simulink model "PMSG_WECS_blocks"  (R2024b)
settings: Solver=ode4  StartTime=0.0  StopTime=Tend  FixedStep=Ts  RelTol=1e-3
InitFcn:
  | %% Parameters of the Simulink model PMSG_WECS_blocks (run automatically by InitFcn)
  | % Scenario selection (can be set in the Command Window before sim):
  | %   scenario = 'step' | 'nominal' | 'robust' ;  useANN = 1 | 0
  | if ~exist('scenario', 'var'), scenario = 'robust'; end
  | if ~exist('useANN', 'var'),   useANN = 1;         end
  | %% Turbine
  | rho = 1.225;  R = 40;  Pn = 2e6;  Wn = 2.23;  Tn = Pn/Wn;
  | J = 2.8e6;  B = 1e3;  lopt = 8.1;  vn = Wn*R/lopt;
  | lam_tab = linspace(1, 16, 301);
  | li_tab  = 1./(1./lam_tab - 0.035);
  | cp_tab  = max(0.5176*(116./li_tab - 5).*exp(-21./li_tab) + 0.0068*lam_tab, 0);
  | %% PMSG (Hasan & Shatil, AJSE 2021, Table I)
  | p = 26;  Rs = 0.78e-3;  Ls = 1.57e-3;  psi = 9.18;
  | %% DC link, filter, grid
  | C = 20e-3;  Vdcr = 1200;  Vgm = 690*sqrt(2/3);  wg = 2*pi*50;
  | Lf = 0.15e-3;  Rf = 2e-3;  fsw = 2160;
  | In = Pn/(1.5*Vgm);  Temax = 1.2*Tn;  Igmax = 1.3*In;  Wmin = 0.5*Wn;  Wmax = Wn;
  | %% Sampling and simulation
  | Ts = 1/(2*fsw);  Tend = 40;  Tlog = 10*Ts;
  | %% Wind
  | Vm = 8.5;  Aw = [1.5 0.2 0.3];  fw = [0.03 0.16 0.17];
  | sig_t = 0.5;  tau_t = 1.5;  seed = 12345;  tau_a = 1.0;
  | Tn_w = 4*Ts;  an = exp(-Tn_w/tau_t);  gn = sqrt(1 - an^2)*sig_t;
  | %% Control
  | wr = 1;  wW = 2;  k11 = 2*wW;  k12 = wW^2;  wv = 60;  k21 = 2*wv;  k22 = wv^2;
  | wi = 500;  Ra = 2*wi*Ls - Rs;  Ki = wi^2*Ls;  Rb = 2*wi*Lf - Rf;  Kig = wi^2*Lf;
  | taud = 2e-3;  kI = k12*(1 - useANN);
  | [c1g, c2g] = meshgrid(linspace(0.5, 1.1, 5), linspace(0.5, 1.1, 5));
  | c1 = c1g(:);  c2 = c2g(:);  b = 0.15;  Gam = 1e7;  sig = 0.02;
  | %% True plant (robustness scenario: parameter mismatch + 50 % grid voltage dip)
  | kTw = 1;  Jt = J;  Rst = Rs;  Lst = Ls;  psit = psi;  Rft = Rf;  Lft = Lf;  Bt = B;
  | windStep = 0;  v0 = Vm;  kdip = 0;  tdip = 25;  ddip = 0.15;
  | switch scenario
  |   case 'step'
  |     windStep = 1;  v0 = 9;
  |   case 'robust'
  |     kTw = 1.10;  Jt = 1.2*J;  Rst = 1.5*Rs;  Lst = 1.2*Ls;  psit = 0.95*psi;
  |     Rft = 1.5*Rf;  Lft = 1.25*Lf;  kdip = 0.5;
  | end
  | %% Initial equilibrium (MPPT at v0, isd = 0, unity power factor)
  | cpf  = @(l) max(0.5176*(116./(1./(1./l - 0.035)) - 5).*exp(-21./(1./(1./l - 0.035))) + 0.0068*l, 0);
  | aero = @(W, v) 0.5*rho*pi*R^2*cpf(W*R/v)*v^3/W;
  | W0   = min(max(lopt*v0/R, Wmin), Wmax);
  | isq0 = -(kTw*aero(W0, v0) - Bt*W0)/(1.5*p*psit);
  | we0  = p*W0;
  | us0  = [-we0*Lst*isq0; Rst*isq0 + we0*psit];
  | Pdc0 = -1.5*us0(2)*isq0;
  | igd0 = (-Vgm + sqrt(Vgm^2 + 4*Rft*Pdc0/1.5))/(2*Rft);
  | ui0  = [Rft*igd0 + Vgm; wg*Lft*igd0];
  | Te0c = 1.5*p*psi*isq0;
  | zW0  = (B*W0 - aero(W0, v0) - Te0c)/(J*k12) * (1 - useANN);
values from neighbouring files (symbols this model uses):
  useANN = 1 | 0'    [PMSG_WECS_simulink.m]
undefined symbols (not defined in the file or in its folder): DiscIntNeverNeededParam
settings Model: Creator=WINDOWS  LastModifiedBy=WINDOWS

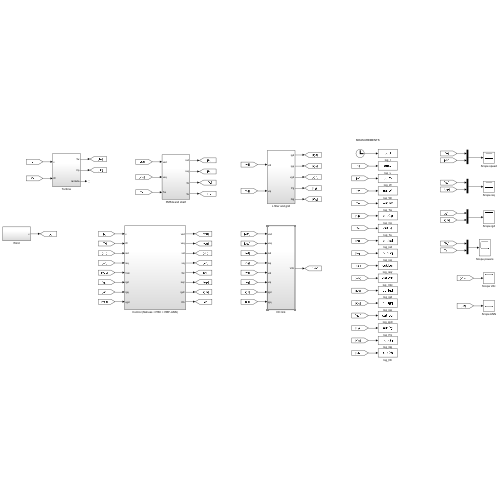
[thumbnail: Simulink's stored preview of the top-level diagram]
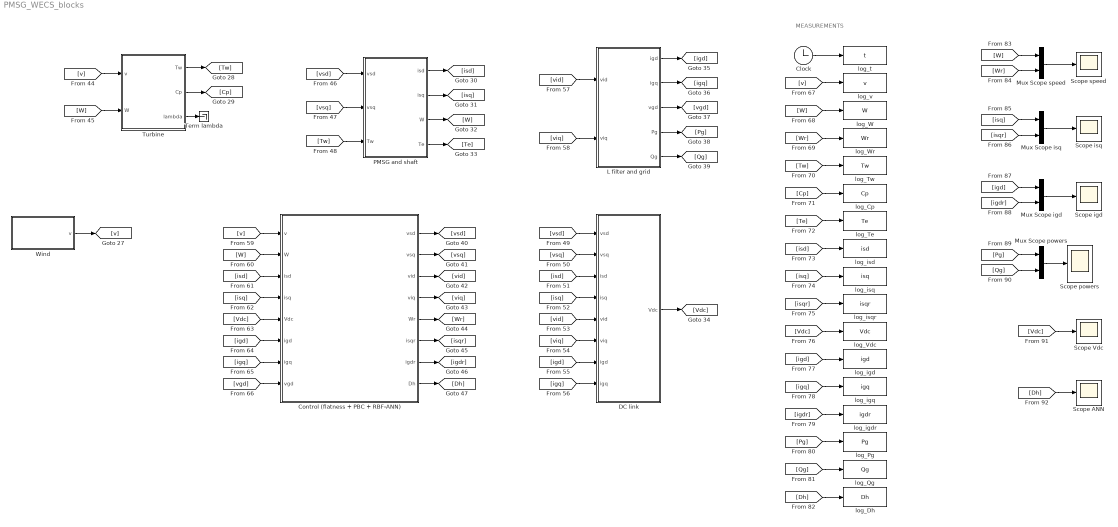
== system PMSG_WECS_blocks ==
  note: MEASUREMENTS
  Clock : Clock
  Control (flatness + PBC + RBF-ANN) : Subsystem
  DC link : Subsystem
  L filter and grid : Subsystem
  Mux Scope igd : Mux  Inputs=2
  Mux Scope isq : Mux  Inputs=2
  Mux Scope powers : Mux  Inputs=2
  Mux Scope speed : Mux  Inputs=2
  PMSG and shaft : Subsystem
  Scope ANN : Scope
  Scope Vdc : Scope
  Scope igd : Scope
  Scope isq : Scope
  Scope powers : Scope
  Scope speed : Scope
  Term lambda : Terminator
  Turbine : Subsystem
  Wind : Subsystem
  log_Cp : ToWorkspace  VariableName=Cp  SampleTime=Tlog
  log_Dh : ToWorkspace  VariableName=Dh  SampleTime=Tlog
  log_Pg : ToWorkspace  VariableName=Pg  SampleTime=Tlog
  log_Qg : ToWorkspace  VariableName=Qg  SampleTime=Tlog
  log_Te : ToWorkspace  VariableName=Te  SampleTime=Tlog
  log_Tw : ToWorkspace  VariableName=Tw  SampleTime=Tlog
  log_Vdc : ToWorkspace  VariableName=Vdc  SampleTime=Tlog
  log_W : ToWorkspace  VariableName=W  SampleTime=Tlog
  log_Wr : ToWorkspace  VariableName=Wr  SampleTime=Tlog
  log_igd : ToWorkspace  VariableName=igd  SampleTime=Tlog
  log_igdr : ToWorkspace  VariableName=igdr  SampleTime=Tlog
  log_igq : ToWorkspace  VariableName=igq  SampleTime=Tlog
  log_isd : ToWorkspace  VariableName=isd  SampleTime=Tlog
  log_isq : ToWorkspace  VariableName=isq  SampleTime=Tlog
  log_isqr : ToWorkspace  VariableName=isqr  SampleTime=Tlog
  log_t : ToWorkspace  VariableName=t  SampleTime=Tlog
  log_v : ToWorkspace  VariableName=v  SampleTime=Tlog
  wires:
  Wind/1(v) -> [v]
  Turbine/1(Tw) -> [Tw]
  Turbine/2(Cp) -> [Cp]
  PMSG and shaft/1(isd) -> [isd]
  PMSG and shaft/2(isq) -> [isq]
  PMSG and shaft/3(W) -> [W]
  PMSG and shaft/4(Te) -> [Te]
  DC link/1(Vdc) -> [Vdc]
  L filter and grid/1(igd) -> [igd]
  L filter and grid/2(igq) -> [igq]
  L filter and grid/3(vgd) -> [vgd]
  L filter and grid/4(Pg) -> [Pg]
  L filter and grid/5(Qg) -> [Qg]
  Control (flatness + PBC + RBF-ANN)/1(vsd) -> [vsd]
  Control (flatness + PBC + RBF-ANN)/2(vsq) -> [vsq]
  Control (flatness + PBC + RBF-ANN)/3(vid) -> [vid]
  Control (flatness + PBC + RBF-ANN)/4(viq) -> [viq]
  Control (flatness + PBC + RBF-ANN)/5(Wr) -> [Wr]
  Control (flatness + PBC + RBF-ANN)/6(isqr) -> [isqr]
  Control (flatness + PBC + RBF-ANN)/7(igdr) -> [igdr]
  Control (flatness + PBC + RBF-ANN)/8(Dh) -> [Dh]
  Turbine/3(lambda) -> Term lambda/1
  [v] -> Turbine/1(v)
  [W] -> Turbine/2(W)
  [vsd] -> PMSG and shaft/1(vsd)
  [vsq] -> PMSG and shaft/2(vsq)
  [Tw] -> PMSG and shaft/3(Tw)
  [vsd] -> DC link/1(vsd)
  [vsq] -> DC link/2(vsq)
  [isd] -> DC link/3(isd)
  [isq] -> DC link/4(isq)
  [vid] -> DC link/5(vid)
  [viq] -> DC link/6(viq)
  [igd] -> DC link/7(igd)
  [igq] -> DC link/8(igq)
  [vid] -> L filter and grid/1(vid)
  [viq] -> L filter and grid/2(viq)
  [v] -> Control (flatness + PBC + RBF-ANN)/1(v)
  [W] -> Control (flatness + PBC + RBF-ANN)/2(W)
  [isd] -> Control (flatness + PBC + RBF-ANN)/3(isd)
  [isq] -> Control (flatness + PBC + RBF-ANN)/4(isq)
  [Vdc] -> Control (flatness + PBC + RBF-ANN)/5(Vdc)
  [igd] -> Control (flatness + PBC + RBF-ANN)/6(igd)
  [igq] -> Control (flatness + PBC + RBF-ANN)/7(igq)
  [vgd] -> Control (flatness + PBC + RBF-ANN)/8(vgd)
  Clock/1 -> log_t/1
  [v] -> log_v/1
  [W] -> log_W/1
  [Wr] -> log_Wr/1
  [Tw] -> log_Tw/1
  [Cp] -> log_Cp/1
  [Te] -> log_Te/1
  [isd] -> log_isd/1
  [isq] -> log_isq/1
  [isqr] -> log_isqr/1
  [Vdc] -> log_Vdc/1
  [igd] -> log_igd/1
  [igq] -> log_igq/1
  [igdr] -> log_igdr/1
  [Pg] -> log_Pg/1
  [Qg] -> log_Qg/1
  [Dh] -> log_Dh/1
  [W] -> Mux Scope speed/1
  [Wr] -> Mux Scope speed/2
  Mux Scope speed/1 -> Scope speed/1
  [isq] -> Mux Scope isq/1
  [isqr] -> Mux Scope isq/2
  Mux Scope isq/1 -> Scope isq/1
  [igd] -> Mux Scope igd/1
  [igdr] -> Mux Scope igd/2
  Mux Scope igd/1 -> Scope igd/1
  [Pg] -> Mux Scope powers/1
  [Qg] -> Mux Scope powers/2
  Mux Scope powers/1 -> Scope powers/1
  [Vdc] -> Scope Vdc/1
  [Dh] -> Scope ANN/1

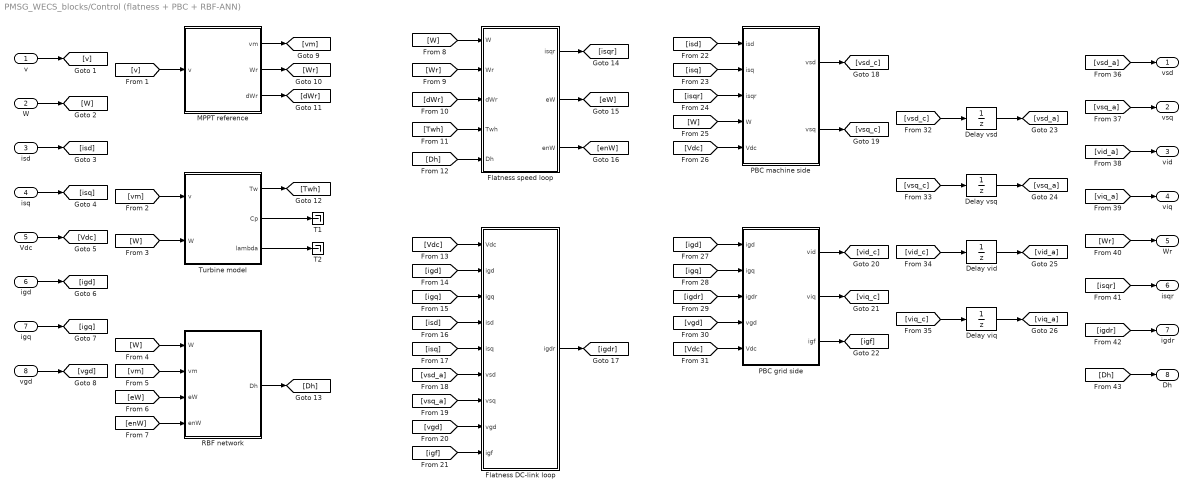
== system PMSG_WECS_blocks/Control (flatness + PBC + RBF-ANN) ==
  v : Inport
  W : Inport  Port=2
  isd : Inport  Port=3
  isq : Inport  Port=4
  Vdc : Inport  Port=5
  igd : Inport  Port=6
  igq : Inport  Port=7
  vgd : Inport  Port=8
  Delay vid : UnitDelay  InitialCondition=ui0(1)  SampleTime=Ts  HasFrameUpgradeWarning=on
  Delay viq : UnitDelay  InitialCondition=ui0(2)  SampleTime=Ts  HasFrameUpgradeWarning=on
  Delay vsd : UnitDelay  InitialCondition=us0(1)  SampleTime=Ts  HasFrameUpgradeWarning=on
  Delay vsq : UnitDelay  InitialCondition=us0(2)  SampleTime=Ts  HasFrameUpgradeWarning=on
  Flatness DC-link loop : Subsystem
  Flatness speed loop : Subsystem
  MPPT reference : Subsystem
  PBC grid side : Subsystem
  PBC machine side : Subsystem
  RBF network : Subsystem
  T1 : Terminator
  T2 : Terminator
  Turbine model : Subsystem
  vsd : Outport
  vsq : Outport  Port=2
  vid : Outport  Port=3
  viq : Outport  Port=4
  Wr : Outport  Port=5
  isqr : Outport  Port=6
  igdr : Outport  Port=7
  Dh : Outport  Port=8
  wires:
  Turbine model/2(Cp) -> T1/1
  Turbine model/3(lambda) -> T2/1
  v/1 -> [v]
  W/1 -> [W]
  isd/1 -> [isd]
  isq/1 -> [isq]
  Vdc/1 -> [Vdc]
  igd/1 -> [igd]
  igq/1 -> [igq]
  vgd/1 -> [vgd]
  MPPT reference/1(vm) -> [vm]
  MPPT reference/2(Wr) -> [Wr]
  MPPT reference/3(dWr) -> [dWr]
  Turbine model/1(Tw) -> [Twh]
  RBF network/1(Dh) -> [Dh]
  Flatness speed loop/1(isqr) -> [isqr]
  Flatness speed loop/2(eW) -> [eW]
  Flatness speed loop/3(enW) -> [enW]
  Flatness DC-link loop/1(igdr) -> [igdr]
  PBC machine side/1(vsd) -> [vsd_c]
  PBC machine side/2(vsq) -> [vsq_c]
  PBC grid side/1(vid) -> [vid_c]
  PBC grid side/2(viq) -> [viq_c]
  PBC grid side/3(igf) -> [igf]
  Delay vsd/1 -> [vsd_a]
  Delay vsq/1 -> [vsq_a]
  Delay vid/1 -> [vid_a]
  Delay viq/1 -> [viq_a]
  [v] -> MPPT reference/1(v)
  [vm] -> Turbine model/1(v)
  [W] -> Turbine model/2(W)
  [W] -> RBF network/1(W)
  [vm] -> RBF network/2(vm)
  [eW] -> RBF network/3(eW)
  [enW] -> RBF network/4(enW)
  [W] -> Flatness speed loop/1(W)
  [Wr] -> Flatness speed loop/2(Wr)
  [dWr] -> Flatness speed loop/3(dWr)
  [Twh] -> Flatness speed loop/4(Twh)
  [Dh] -> Flatness speed loop/5(Dh)
  [Vdc] -> Flatness DC-link loop/1(Vdc)
  [igd] -> Flatness DC-link loop/2(igd)
  [igq] -> Flatness DC-link loop/3(igq)
  [isd] -> Flatness DC-link loop/4(isd)
  [isq] -> Flatness DC-link loop/5(isq)
  [vsd_a] -> Flatness DC-link loop/6(vsd)
  [vsq_a] -> Flatness DC-link loop/7(vsq)
  [vgd] -> Flatness DC-link loop/8(vgd)
  [igf] -> Flatness DC-link loop/9(igf)
  [isd] -> PBC machine side/1(isd)
  [isq] -> PBC machine side/2(isq)
  [isqr] -> PBC machine side/3(isqr)
  [W] -> PBC machine side/4(W)
  [Vdc] -> PBC machine side/5(Vdc)
  [igd] -> PBC grid side/1(igd)
  [igq] -> PBC grid side/2(igq)
  [igdr] -> PBC grid side/3(igdr)
  [vgd] -> PBC grid side/4(vgd)
  [Vdc] -> PBC grid side/5(Vdc)
  [vsd_c] -> Delay vsd/1
  [vsq_c] -> Delay vsq/1
  [vid_c] -> Delay vid/1
  [viq_c] -> Delay viq/1
  [vsd_a] -> vsd/1
  [vsq_a] -> vsq/1
  [vid_a] -> vid/1
  [viq_a] -> viq/1
  [Wr] -> Wr/1
  [isqr] -> isqr/1
  [igdr] -> igdr/1
  [Dh] -> Dh/1

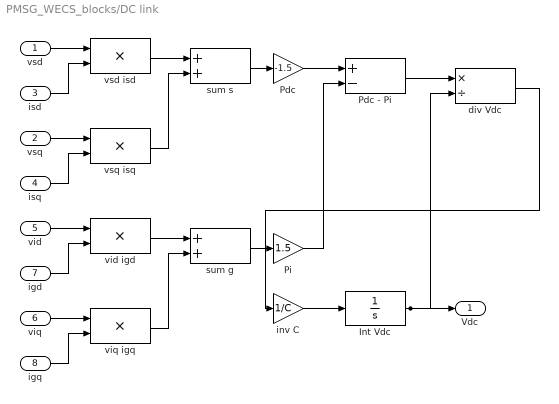
== system PMSG_WECS_blocks/DC link ==
  vsd : Inport
  vsq : Inport  Port=2
  isd : Inport  Port=3
  isq : Inport  Port=4
  vid : Inport  Port=5
  viq : Inport  Port=6
  igd : Inport  Port=7
  igq : Inport  Port=8
  Int Vdc : Integrator  InitialCondition=Vdcr
  Pdc : Gain  Gain=-1.5
  Pdc - Pi : Sum  Inputs=+-
  Pi : Gain  Gain=1.5
  div Vdc : Product  Inputs=*/
  inv C : Gain  Gain=1/C
  sum g : Sum
  sum s : Sum
  vid igd : Product  Inputs=**
  viq igq : Product  Inputs=**
  vsd isd : Product  Inputs=**
  vsq isq : Product  Inputs=**
  Vdc : Outport
  wires:
  vsd/1 -> vsd isd/1
  isd/1 -> vsd isd/2
  vsq/1 -> vsq isq/1
  isq/1 -> vsq isq/2
  viq/1 -> viq igq/1
  vid/1 -> vid igd/1
  igd/1 -> vid igd/2
  igq/1 -> viq igq/2
  vsq isq/1 -> sum s/2
  vsd isd/1 -> sum s/1
  viq igq/1 -> sum g/2
  vid igd/1 -> sum g/1
  sum s/1 -> Pdc/1
  sum g/1 -> Pi/1
  Pdc/1 -> Pdc - Pi/1
  Pi/1 -> Pdc - Pi/2
  inv C/1 -> Int Vdc/1
  Pdc - Pi/1 -> div Vdc/1
  div Vdc/1 -> inv C/1
  Int Vdc/1 -> div Vdc/2, Vdc/1

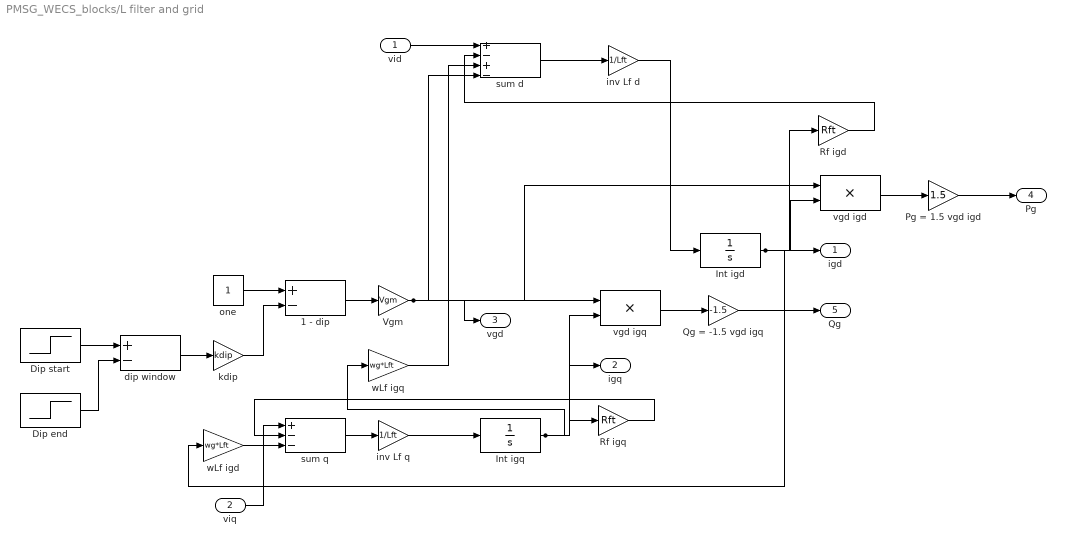
== system PMSG_WECS_blocks/L filter and grid ==
  vid : Inport
  viq : Inport  Port=2
  1 - dip : Sum  Inputs=+-
  Dip end : Step  Time=tdip+ddip  SampleTime=0
  Dip start : Step  Time=tdip  SampleTime=0
  Int igd : Integrator  InitialCondition=igd0
  Int igq : Integrator
  Pg = 1.5 vgd igd : Gain  Gain=1.5
  Qg = -1.5 vgd igq : Gain  Gain=-1.5
  Rf igd : Gain  Gain=Rft
  Rf igq : Gain  Gain=Rft
  Vgm : Gain  Gain=Vgm
  dip window : Sum  Inputs=+-
  inv Lf d : Gain  Gain=1/Lft
  inv Lf q : Gain  Gain=1/Lft
  kdip : Gain  Gain=kdip
  one : Constant
  sum d : Sum  Inputs=+-+-
  sum q : Sum  Inputs=+--
  vgd igd : Product  Inputs=**
  vgd igq : Product  Inputs=**
  wLf igd : Gain  Gain=wg*Lft
  wLf igq : Gain  Gain=wg*Lft
  igd : Outport
  igq : Outport  Port=2
  vgd : Outport  Port=3
  Pg : Outport  Port=4
  Qg : Outport  Port=5
  wires:
  sum q/1 -> inv Lf q/1
  wLf igd/1 -> sum q/3
  Dip start/1 -> dip window/1
  Dip end/1 -> dip window/2
  viq/1 -> sum q/1
  kdip/1 -> 1 - dip/2
  dip window/1 -> kdip/1
  one/1 -> 1 - dip/1
  1 - dip/1 -> Vgm/1
  vid/1 -> sum d/1
  Vgm/1 -> vgd igq/1, vgd/1, sum d/4, vgd igd/1
  sum d/1 -> inv Lf d/1
  wLf igq/1 -> sum d/3
  inv Lf q/1 -> Int igq/1
  Int igq/1 -> wLf igq/1, Rf igq/1, vgd igq/2, igq/1
  inv Lf d/1 -> Int igd/1
  vgd igq/1 -> Qg = -1.5 vgd igq/1
  Rf igq/1 -> sum q/2
  Int igd/1 -> wLf igd/1, Rf igd/1, vgd igd/2, igd/1
  Qg = -1.5 vgd igq/1 -> Qg/1
  Rf igd/1 -> sum d/2
  vgd igd/1 -> Pg = 1.5 vgd igd/1
  Pg = 1.5 vgd igd/1 -> Pg/1

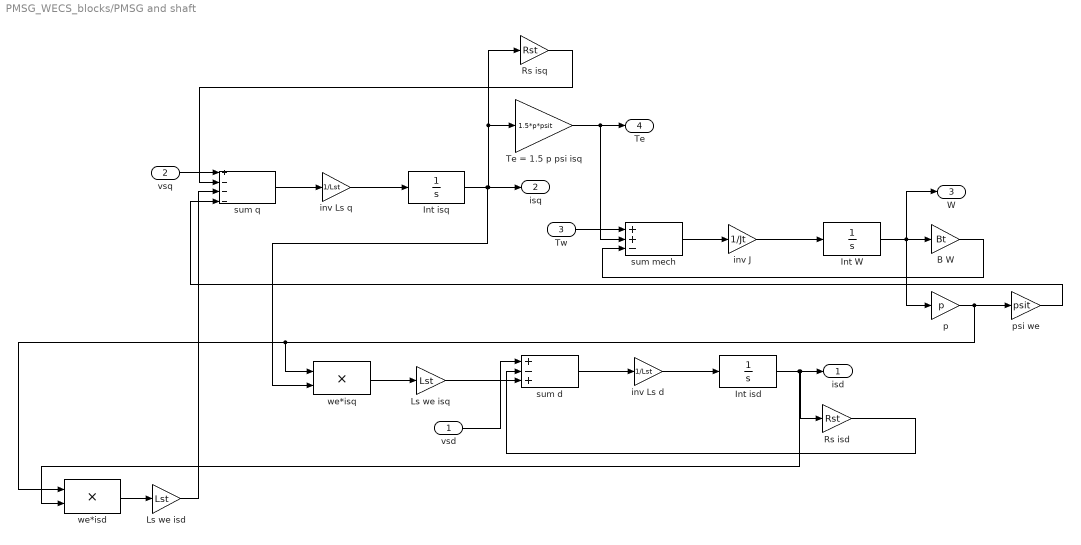
== system PMSG_WECS_blocks/PMSG and shaft ==
  vsd : Inport
  vsq : Inport  Port=2
  Tw : Inport  Port=3
  B W : Gain  Gain=Bt
  Int W : Integrator  InitialCondition=W0
  Int isd : Integrator
  Int isq : Integrator  InitialCondition=isq0
  Ls we isd : Gain  Gain=Lst
  Ls we isq : Gain  Gain=Lst
  Rs isd : Gain  Gain=Rst
  Rs isq : Gain  Gain=Rst
  Te = 1.5 p psi isq : Gain  Gain=1.5*p*psit
  inv J : Gain  Gain=1/Jt
  inv Ls d : Gain  Gain=1/Lst
  inv Ls q : Gain  Gain=1/Lst
  p : Gain  Gain=p
  psi we : Gain  Gain=psit
  sum d : Sum  Inputs=+-+
  sum mech : Sum  Inputs=++-
  sum q : Sum  Inputs=+---
  we*isd : Product  Inputs=**
  we*isq : Product  Inputs=**
  isd : Outport
  isq : Outport  Port=2
  W : Outport  Port=3
  Te : Outport  Port=4
  wires:
  Int isq/1 -> Te = 1.5 p psi isq/1, Rs isq/1, isq/1, we*isq/2
  Int W/1 -> p/1, B W/1, W/1
  Int isd/1 -> Rs isd/1, isd/1, we*isd/2
  we*isd/1 -> Ls we isd/1
  vsq/1 -> sum q/1
  sum q/1 -> inv Ls q/1
  Ls we isd/1 -> sum q/3
  inv Ls q/1 -> Int isq/1
  Ls we isq/1 -> sum d/3
  we*isq/1 -> Ls we isq/1
  vsd/1 -> sum d/1
  Rs isq/1 -> sum q/2
  Te = 1.5 p psi isq/1 -> sum mech/2, Te/1
  Tw/1 -> sum mech/1
  sum d/1 -> inv Ls d/1
  inv J/1 -> Int W/1
  sum mech/1 -> inv J/1
  inv Ls d/1 -> Int isd/1
  Rs isd/1 -> sum d/2
  B W/1 -> sum mech/3
  p/1 -> we*isq/1, we*isd/1, psi we/1
  psi we/1 -> sum q/4

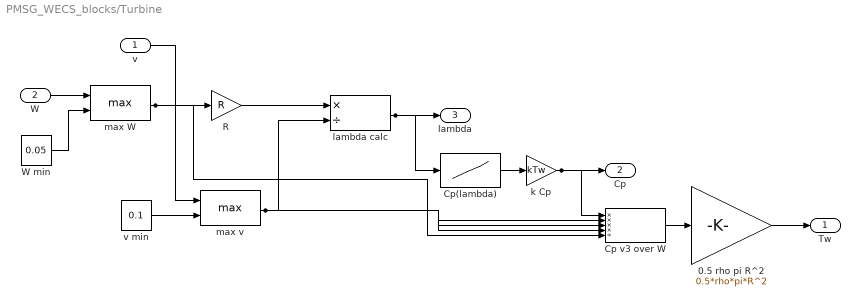
== system PMSG_WECS_blocks/Turbine ==
  v : Inport
  W : Inport  Port=2
  0.5 rho pi R^2 : Gain  Gain=0.5*rho*pi*R^2
  Cp v3 over W : Product  Inputs=****/
  Cp(lambda) : Lookup_n-D  NumberOfTableDimensions=1  BreakpointsForDimension1=lam_tab  Table=cp_tab  ExtrapMethod=Clip  InternalRulePriority=Speed  RndMeth=Simplest
  R : Gain  Gain=R
  W min : Constant  Value=0.05
  k Cp : Gain  Gain=kTw
  lambda calc : Product  Inputs=*/
  max W : MinMax  Function=max  Inputs=2
  max v : MinMax  Function=max  Inputs=2
  v min : Constant  Value=0.1
  Tw : Outport
  Cp : Outport  Port=2
  lambda : Outport  Port=3
  wires:
  W/1 -> max W/1
  lambda calc/1 -> lambda/1, Cp(lambda)/1
  W min/1 -> max W/2
  v min/1 -> max v/2
  v/1 -> max v/1
  max W/1 -> Cp v3 over W/5, R/1
  R/1 -> lambda calc/1
  max v/1 -> Cp v3 over W/2, Cp v3 over W/4, lambda calc/2, Cp v3 over W/3
  Cp(lambda)/1 -> k Cp/1
  k Cp/1 -> Cp/1, Cp v3 over W/1
  Cp v3 over W/1 -> 0.5 rho pi R^2/1
  0.5 rho pi R^2/1 -> Tw/1

== system PMSG_WECS_blocks/Wind ==
  Harmonic 1 : Sin  Amplitude=Aw(1)  Frequency=2*pi*fw(1)  SampleTime=0
  Harmonic 2 : Sin  Amplitude=Aw(2)  Frequency=2*pi*fw(2)  SampleTime=0
  Harmonic 3 : Sin  Amplitude=Aw(3)  Frequency=2*pi*fw(3)  SampleTime=0
  Profile : Switch  Criteria=u2 > Threshold  Threshold=0.5  SaturateOnIntegerOverflow=off  InputSameDT=off
  Step 10 s : Step  Time=10  After=2  SampleTime=0
  Step 25 s : Step  Time=25  After=-3  SampleTime=0
  Step wind : Sum  Inputs=+++
  Turbulence AR1 : DiscreteTransferFcn  Numerator=[gn 0]  Denominator=[1 -an]  SampleTime=Tn_w
  Turbulent wind : Sum  Inputs=+++++
  Vm : Constant  Value=Vm
  White noise : RandomNumber  Seed=seed  SampleTime=Tn_w
  v base : Constant  Value=9
  windStep : Constant  Value=windStep
  v : Outport
  wires:
  v base/1 -> Step wind/1
  White noise/1 -> Turbulence AR1/1
  Step 10 s/1 -> Step wind/2
  Harmonic 3/1 -> Turbulent wind/4
  Harmonic 1/1 -> Turbulent wind/2
  Vm/1 -> Turbulent wind/1
  Step 25 s/1 -> Step wind/3
  Harmonic 2/1 -> Turbulent wind/3
  Turbulence AR1/1 -> Turbulent wind/5
  Step wind/1 -> Profile/1
  windStep/1 -> Profile/2
  Turbulent wind/1 -> Profile/3
  Profile/1 -> v/1

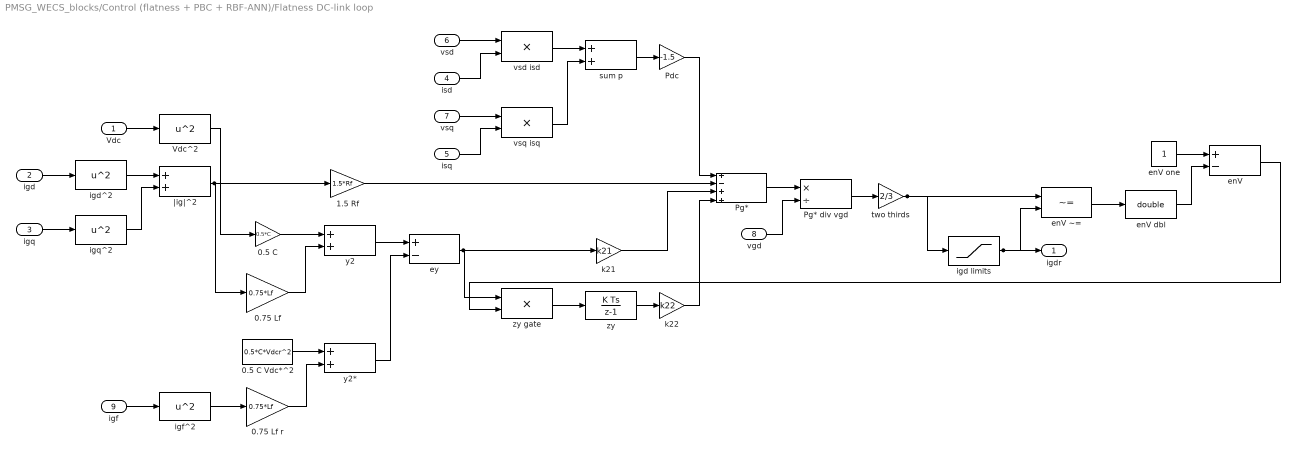
== system PMSG_WECS_blocks/Control (flatness + PBC + RBF-ANN)/Flatness DC-link loop ==
  Vdc : Inport
  igd : Inport  Port=2
  igq : Inport  Port=3
  isd : Inport  Port=4
  isq : Inport  Port=5
  vsd : Inport  Port=6
  vsq : Inport  Port=7
  vgd : Inport  Port=8
  igf : Inport  Port=9
  0.5 C : Gain  Gain=0.5*C
  0.5 C Vdc*^2 : Constant  Value=0.5*C*Vdcr^2
  0.75 Lf : Gain  Gain=0.75*Lf
  0.75 Lf r : Gain  Gain=0.75*Lf
  1.5 Rf : Gain  Gain=1.5*Rf
  Pdc : Gain  Gain=-1.5
  Pg* : Sum  Inputs=+-++
  Pg* div vgd : Product  Inputs=*/
  Vdc^2 : Math  Operator=square
  enV : Sum  Inputs=+-
  enV dbl : DataTypeConversion  OutDataTypeStr=double  SaturateOnIntegerOverflow=off  RndMeth=Floor
  enV one : Constant
  enV ~= : RelationalOperator  Operator=~=  OutDataTypeStr=boolean  RndMeth=Simplest  InputSameDT=off
  ey : Sum  Inputs=+-
  igd limits : Saturate  UpperLimit=Igmax  LowerLimit=-Igmax
  igd^2 : Math  Operator=square
  igf^2 : Math  Operator=square
  igq^2 : Math  Operator=square
  k21 : Gain  Gain=k21
  k22 : Gain  Gain=k22
  sum p : Sum
  two thirds : Gain  Gain=2/3
  vsd isd : Product  Inputs=**
  vsq isq : Product  Inputs=**
  y2 : Sum
  y2* : Sum
  zy : DiscreteIntegrator  SampleTime=Ts  ICPrevOutput=DiscIntNeverNeededParam  ICPrevScaledInput=DiscIntNeverNeededParam
  zy gate : Product  Inputs=**
  |ig|^2 : Sum
  igdr : Outport
  wires:
  isq/1 -> vsq isq/2
  igd/1 -> igd^2/1
  igq/1 -> igq^2/1
  igf/1 -> igf^2/1
  Vdc/1 -> Vdc^2/1
  igq^2/1 -> |ig|^2/2
  igd^2/1 -> |ig|^2/1
  Vdc^2/1 -> 0.5 C/1
  |ig|^2/1 -> 1.5 Rf/1, 0.75 Lf/1
  igf^2/1 -> 0.75 Lf r/1
  0.5 C/1 -> y2/1
  y2/1 -> ey/1
  0.75 Lf/1 -> y2/2
  y2*/1 -> ey/2
  0.5 C Vdc*^2/1 -> y2*/1
  isd/1 -> vsd isd/2
  0.75 Lf r/1 -> y2*/2
  Pg*/1 -> Pg* div vgd/1
  1.5 Rf/1 -> Pg*/2
  Pdc/1 -> Pg*/1
  vsd/1 -> vsd isd/1
  vsq/1 -> vsq isq/1
  ey/1 -> k21/1, zy gate/1
  zy gate/1 -> zy/1
  vsd isd/1 -> sum p/1
  vsq isq/1 -> sum p/2
  sum p/1 -> Pdc/1
  k21/1 -> Pg*/3
  enV ~=/1 -> enV dbl/1
  zy/1 -> k22/1
  k22/1 -> Pg*/4
  vgd/1 -> Pg* div vgd/2
  Pg* div vgd/1 -> two thirds/1
  two thirds/1 -> igd limits/1, enV ~=/1
  igd limits/1 -> enV ~=/2, igdr/1
  enV dbl/1 -> enV/2
  enV one/1 -> enV/1
  enV/1 -> zy gate/2

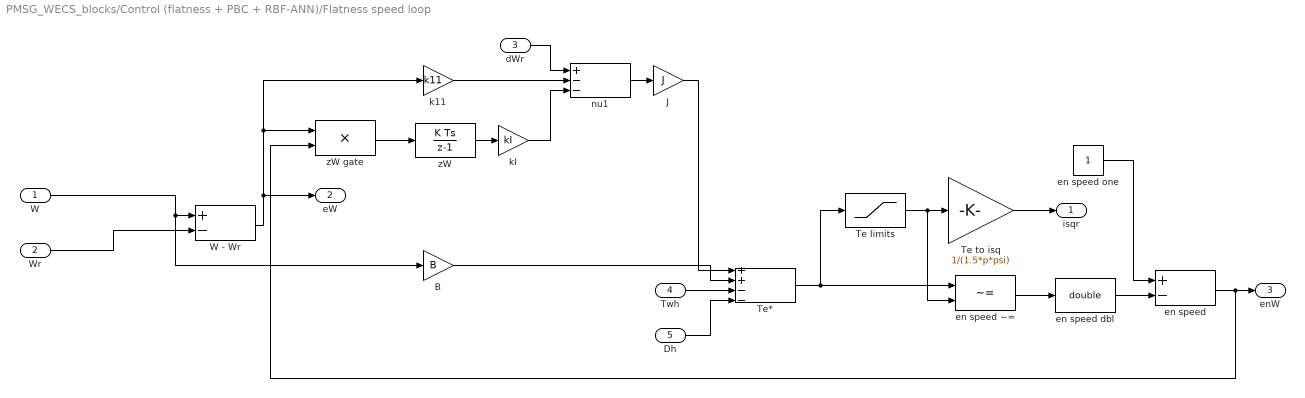
== system PMSG_WECS_blocks/Control (flatness + PBC + RBF-ANN)/Flatness speed loop ==
  W : Inport
  Wr : Inport  Port=2
  dWr : Inport  Port=3
  Twh : Inport  Port=4
  Dh : Inport  Port=5
  B : Gain  Gain=B
  J : Gain  Gain=J
  Te limits : Saturate  UpperLimit=0  LowerLimit=-Temax
  Te to isq : Gain  Gain=1/(1.5*p*psi)
  Te* : Sum  Inputs=++--
  W - Wr : Sum  Inputs=+-
  en speed : Sum  Inputs=+-
  en speed dbl : DataTypeConversion  OutDataTypeStr=double  SaturateOnIntegerOverflow=off  RndMeth=Floor
  en speed one : Constant
  en speed ~= : RelationalOperator  Operator=~=  OutDataTypeStr=boolean  RndMeth=Simplest  InputSameDT=off
  k11 : Gain  Gain=k11
  kI : Gain  Gain=kI
  nu1 : Sum  Inputs=+--
  zW : DiscreteIntegrator  InitialCondition=zW0  SampleTime=Ts  ICPrevOutput=DiscIntNeverNeededParam  ICPrevScaledInput=DiscIntNeverNeededParam
  zW gate : Product  Inputs=**
  isqr : Outport
  eW : Outport  Port=2
  enW : Outport  Port=3
  wires:
  Dh/1 -> Te*/4
  W/1 -> B/1, W - Wr/1
  dWr/1 -> nu1/1
  W - Wr/1 -> k11/1, zW gate/1, eW/1
  Wr/1 -> W - Wr/2
  zW/1 -> kI/1
  zW gate/1 -> zW/1
  k11/1 -> nu1/2
  B/1 -> Te*/2
  kI/1 -> nu1/3
  nu1/1 -> J/1
  J/1 -> Te*/1
  Twh/1 -> Te*/3
  Te*/1 -> en speed ~=/1, Te limits/1
  Te limits/1 -> en speed ~=/2, Te to isq/1
  Te to isq/1 -> isqr/1
  en speed dbl/1 -> en speed/2
  en speed ~=/1 -> en speed dbl/1
  en speed/1 -> zW gate/2, enW/1
  en speed one/1 -> en speed/1

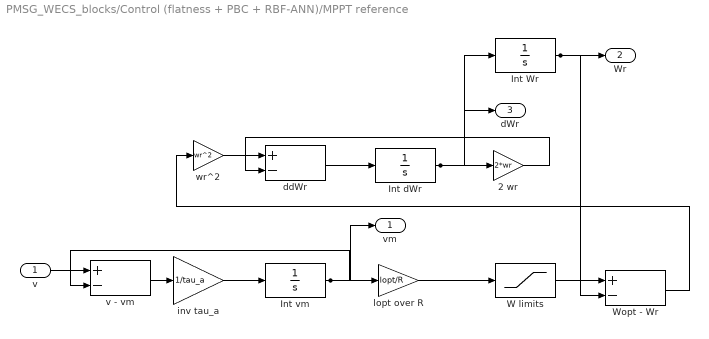
== system PMSG_WECS_blocks/Control (flatness + PBC + RBF-ANN)/MPPT reference ==
  v : Inport
  2 wr : Gain  Gain=2*wr
  Int Wr : Integrator  InitialCondition=W0
  Int dWr : Integrator
  Int vm : Integrator  InitialCondition=v0
  W limits : Saturate  UpperLimit=Wmax  LowerLimit=Wmin
  Wopt - Wr : Sum  Inputs=+-
  ddWr : Sum  Inputs=+-
  inv tau_a : Gain  Gain=1/tau_a
  lopt over R : Gain  Gain=lopt/R
  v - vm : Sum  Inputs=+-
  wr^2 : Gain  Gain=wr^2
  vm : Outport
  Wr : Outport  Port=2
  dWr : Outport  Port=3
  wires:
  W limits/1 -> Wopt - Wr/1
  v/1 -> v - vm/1
  inv tau_a/1 -> Int vm/1
  v - vm/1 -> inv tau_a/1
  wr^2/1 -> ddWr/1
  ddWr/1 -> Int dWr/1
  Int vm/1 -> lopt over R/1, vm/1, v - vm/2
  Int dWr/1 -> 2 wr/1, Int Wr/1, dWr/1
  lopt over R/1 -> W limits/1
  Int Wr/1 -> Wr/1, Wopt - Wr/2
  Wopt - Wr/1 -> wr^2/1
  2 wr/1 -> ddWr/2

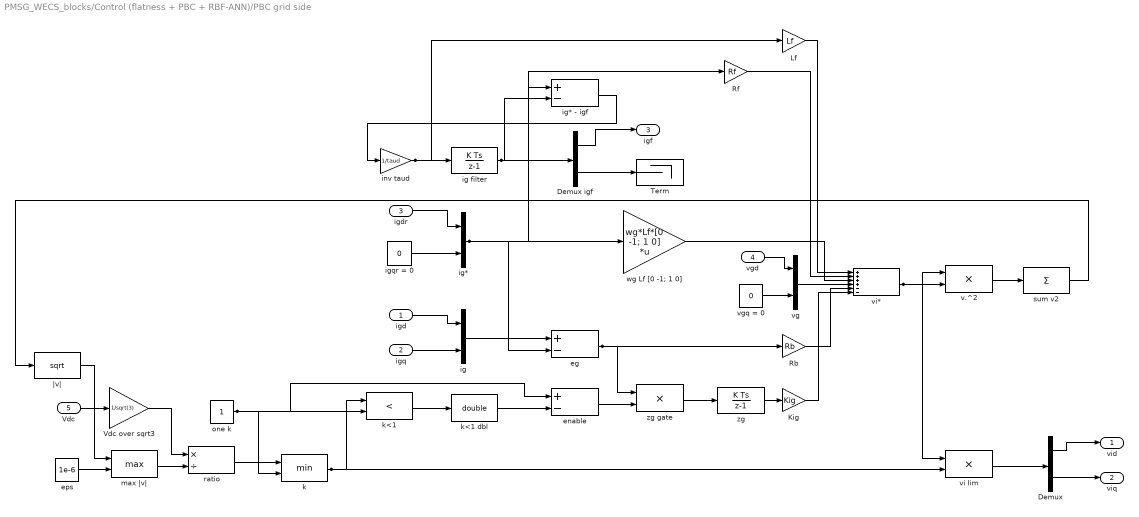
== system PMSG_WECS_blocks/Control (flatness + PBC + RBF-ANN)/PBC grid side ==
  igd : Inport
  igq : Inport  Port=2
  igdr : Inport  Port=3
  vgd : Inport  Port=4
  Vdc : Inport  Port=5
  Demux : Demux  Outputs=2
  Demux igf : Demux  Outputs=2
  Kig : Gain  Gain=Kig
  Lf : Gain  Gain=Lf
  Rb : Gain  Gain=Rb
  Rf : Gain  Gain=Rf
  Term : Terminator
  Vdc over sqrt3 : Gain  Gain=1/sqrt(3)
  eg : Sum  Inputs=+-
  enable : Sum  Inputs=+-
  eps : Constant  Value=1e-6
  ig : Mux  Inputs=2
  ig filter : DiscreteIntegrator  InitialCondition=[igd0; 0]  SampleTime=Ts  ICPrevOutput=DiscIntNeverNeededParam  ICPrevScaledInput=DiscIntNeverNeededParam
  ig* : Mux  Inputs=2
  ig* - igf : Sum  Inputs=+-
  igqr = 0 : Constant  Value=0
  inv taud : Gain  Gain=1/taud
  k : MinMax  Inputs=2
  k<1 : RelationalOperator  Operator=<  OutDataTypeStr=boolean  RndMeth=Simplest  InputSameDT=off
  k<1 dbl : DataTypeConversion  OutDataTypeStr=double  SaturateOnIntegerOverflow=off  RndMeth=Floor
  max |v| : MinMax  Function=max  Inputs=2
  one k : Constant
  ratio : Product  Inputs=*/
  sum v2 : Sum  Inputs=+
  v.^2 : Product  Inputs=**
  vg : Mux  Inputs=2
  vgq = 0 : Constant  Value=0
  vi lim : Product  Inputs=**
  vi* : Sum  Inputs=++++--
  wg Lf [0 -1; 1 0] : Gain  Gain=wg*Lf*[0 -1; 1 0]  Multiplication=Matrix(K*u)
  zg : DiscreteIntegrator  InitialCondition=[0; 0]  SampleTime=Ts  ICPrevOutput=DiscIntNeverNeededParam  ICPrevScaledInput=DiscIntNeverNeededParam
  zg gate : Product  Inputs=**
  |v| : Sqrt
  vid : Outport
  viq : Outport  Port=2
  igf : Outport  Port=3
  wires:
  |v|/1 -> max |v|/1
  eps/1 -> max |v|/2
  Vdc over sqrt3/1 -> ratio/1
  max |v|/1 -> ratio/2
  ig* - igf/1 -> inv taud/1
  Vdc/1 -> Vdc over sqrt3/1
  v.^2/1 -> sum v2/1
  k/1 -> vi lim/2, k<1/1
  one k/1 -> enable/1, k/2, k<1/2
  ratio/1 -> k/1
  inv taud/1 -> Lf/1, ig filter/1
  ig*/1 -> wg Lf [0 -1; 1 0]/1, Rf/1, ig* - igf/1, eg/2
  igdr/1 -> ig*/1
  vgq = 0/1 -> vg/2
  igqr = 0/1 -> ig*/2
  igd/1 -> ig/1
  igq/1 -> ig/2
  vi lim/1 -> Demux/1
  k<1/1 -> k<1 dbl/1
  ig filter/1 -> ig* - igf/2, Demux igf/1
  sum v2/1 -> |v|/1
  ig/1 -> eg/1
  k<1 dbl/1 -> enable/2
  Demux igf/1 -> igf/1
  Demux igf/2 -> Term/1
  eg/1 -> Rb/1, zg gate/1
  enable/1 -> zg gate/2
  Rf/1 -> vi*/2
  wg Lf [0 -1; 1 0]/1 -> vi*/3
  zg gate/1 -> zg/1
  vgd/1 -> vg/1
  zg/1 -> Kig/1
  Lf/1 -> vi*/1
  vg/1 -> vi*/4
  Rb/1 -> vi*/5
  Kig/1 -> vi*/6
  vi*/1 -> v.^2/1, v.^2/2, vi lim/1
  Demux/1 -> vid/1
  Demux/2 -> viq/1

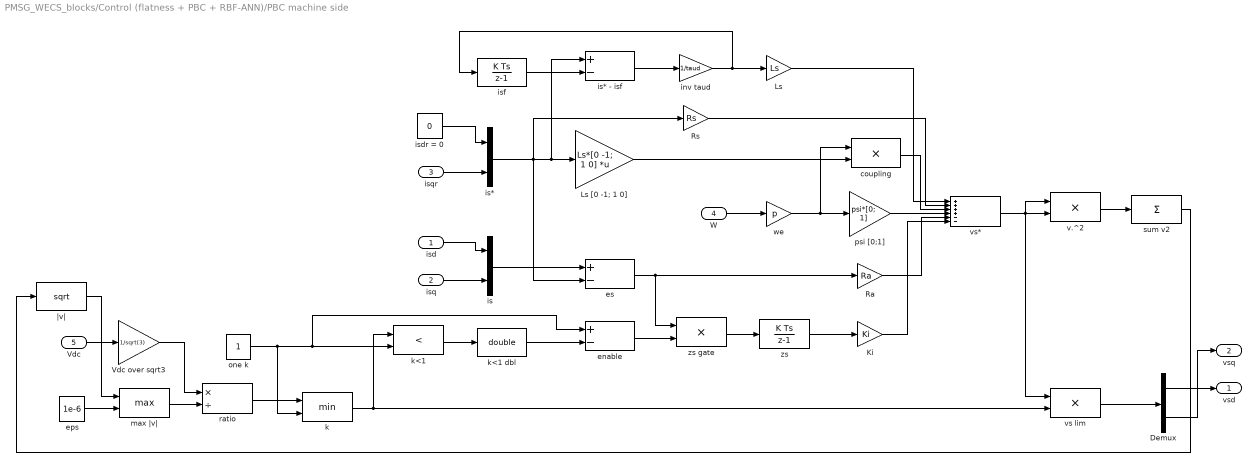
== system PMSG_WECS_blocks/Control (flatness + PBC + RBF-ANN)/PBC machine side ==
  isd : Inport
  isq : Inport  Port=2
  isqr : Inport  Port=3
  W : Inport  Port=4
  Vdc : Inport  Port=5
  Demux : Demux  Outputs=2
  Ki : Gain  Gain=Ki
  Ls : Gain  Gain=Ls
  Ls [0 -1; 1 0] : Gain  Gain=Ls*[0 -1; 1 0]  Multiplication=Matrix(K*u)
  Ra : Gain  Gain=Ra
  Rs : Gain  Gain=Rs
  Vdc over sqrt3 : Gain  Gain=1/sqrt(3)
  coupling : Product  Inputs=**
  enable : Sum  Inputs=+-
  eps : Constant  Value=1e-6
  es : Sum  Inputs=+-
  inv taud : Gain  Gain=1/taud
  is : Mux  Inputs=2
  is* : Mux  Inputs=2
  is* - isf : Sum  Inputs=+-
  isdr = 0 : Constant  Value=0
  isf : DiscreteIntegrator  InitialCondition=[0; isq0]  SampleTime=Ts  ICPrevOutput=DiscIntNeverNeededParam  ICPrevScaledInput=DiscIntNeverNeededParam
  k : MinMax  Inputs=2
  k<1 : RelationalOperator  Operator=<  OutDataTypeStr=boolean  RndMeth=Simplest  InputSameDT=off
  k<1 dbl : DataTypeConversion  OutDataTypeStr=double  SaturateOnIntegerOverflow=off  RndMeth=Floor
  max |v| : MinMax  Function=max  Inputs=2
  one k : Constant
  psi [0;1] : Gain  Gain=psi*[0; 1]
  ratio : Product  Inputs=*/
  sum v2 : Sum  Inputs=+
  v.^2 : Product  Inputs=**
  vs lim : Product  Inputs=**
  vs* : Sum  Inputs=++++--
  we : Gain  Gain=p
  zs : DiscreteIntegrator  InitialCondition=[0; 0]  SampleTime=Ts  ICPrevOutput=DiscIntNeverNeededParam  ICPrevScaledInput=DiscIntNeverNeededParam
  zs gate : Product  Inputs=**
  |v| : Sqrt
  vsd : Outport
  vsq : Outport  Port=2
  wires:
  is* - isf/1 -> inv taud/1
  max |v|/1 -> ratio/2
  |v|/1 -> max |v|/1
  eps/1 -> max |v|/2
  psi [0;1]/1 -> vs*/4
  k/1 -> vs lim/2, k<1/1
  one k/1 -> k<1/2, enable/1, k/2
  Demux/1 -> vsd/1
  Vdc/1 -> Vdc over sqrt3/1
  Vdc over sqrt3/1 -> ratio/1
  ratio/1 -> k/1
  Ra/1 -> vs*/5
  isdr = 0/1 -> is*/1
  isqr/1 -> is*/2
  isd/1 -> is/1
  isq/1 -> is/2
  vs lim/1 -> Demux/1
  k<1/1 -> k<1 dbl/1
  coupling/1 -> vs*/3
  Ls [0 -1; 1 0]/1 -> coupling/2
  isf/1 -> is* - isf/2
  is*/1 -> is* - isf/1, Ls [0 -1; 1 0]/1, Rs/1, es/2
  is/1 -> es/1
  enable/1 -> zs gate/2
  k<1 dbl/1 -> enable/2
  es/1 -> Ra/1, zs gate/1
  inv taud/1 -> isf/1, Ls/1
  Rs/1 -> vs*/2
  W/1 -> we/1
  zs gate/1 -> zs/1
  Ls/1 -> vs*/1
  we/1 -> coupling/1, psi [0;1]/1
  zs/1 -> Ki/1
  Ki/1 -> vs*/6
  Demux/2 -> vsq/1
  vs*/1 -> v.^2/2, vs lim/1, v.^2/1
  sum v2/1 -> |v|/1
  v.^2/1 -> sum v2/1

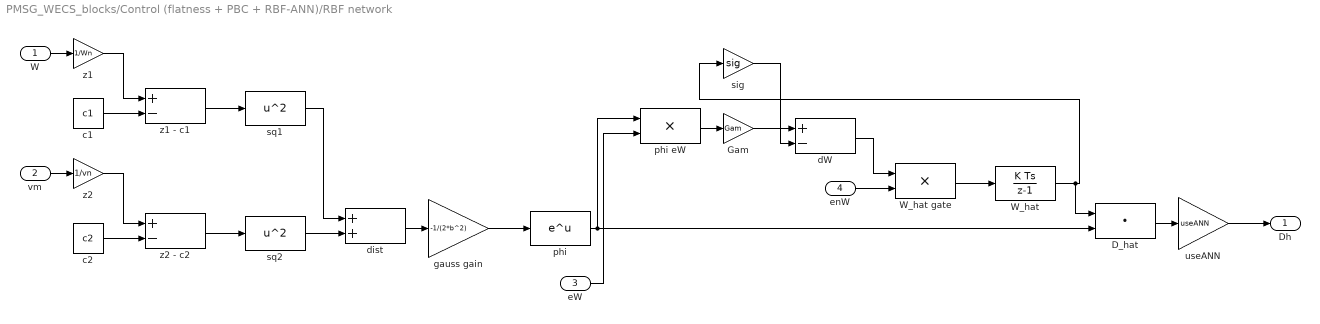
== system PMSG_WECS_blocks/Control (flatness + PBC + RBF-ANN)/RBF network ==
  W : Inport
  vm : Inport  Port=2
  eW : Inport  Port=3
  enW : Inport  Port=4
  D_hat : DotProduct  OutDataTypeStr=Inherit: Inherit via internal rule
  Gam : Gain  Gain=Gam
  W_hat : DiscreteIntegrator  InitialCondition=zeros(25,1)  SampleTime=Ts  ICPrevOutput=DiscIntNeverNeededParam  ICPrevScaledInput=DiscIntNeverNeededParam
  W_hat gate : Product  Inputs=**
  c1 : Constant  Value=c1
  c2 : Constant  Value=c2
  dW : Sum  Inputs=+-
  dist : Sum
  gauss gain : Gain  Gain=-1/(2*b^2)
  phi : Math
  phi eW : Product  Inputs=**
  sig : Gain  Gain=sig
  sq1 : Math  Operator=square
  sq2 : Math  Operator=square
  useANN : Gain  Gain=useANN
  z1 : Gain  Gain=1/Wn
  z1 - c1 : Sum  Inputs=+-
  z2 : Gain  Gain=1/vn
  z2 - c2 : Sum  Inputs=+-
  Dh : Outport
  wires:
  W/1 -> z1/1
  vm/1 -> z2/1
  z2 - c2/1 -> sq2/1
  z1/1 -> z1 - c1/1
  c1/1 -> z1 - c1/2
  z2/1 -> z2 - c2/1
  c2/1 -> z2 - c2/2
  z1 - c1/1 -> sq1/1
  sq1/1 -> dist/1
  dist/1 -> gauss gain/1
  sq2/1 -> dist/2
  gauss gain/1 -> phi/1
  phi/1 -> phi eW/1, D_hat/2
  eW/1 -> phi eW/2
  phi eW/1 -> Gam/1
  dW/1 -> W_hat gate/1
  sig/1 -> dW/2
  Gam/1 -> dW/1
  enW/1 -> W_hat gate/2
  W_hat gate/1 -> W_hat/1
  W_hat/1 -> sig/1, D_hat/1
  D_hat/1 -> useANN/1
  useANN/1 -> Dh/1

== system PMSG_WECS_blocks/Control (flatness + PBC + RBF-ANN)/Turbine model ==
  v : Inport
  W : Inport  Port=2
  0.5 rho pi R^2 : Gain  Gain=0.5*rho*pi*R^2
  Cp v3 over W : Product  Inputs=****/
  Cp(lambda) : Lookup_n-D  NumberOfTableDimensions=1  BreakpointsForDimension1=lam_tab  Table=cp_tab  ExtrapMethod=Clip  InternalRulePriority=Speed  RndMeth=Simplest
  R : Gain  Gain=R
  W min : Constant  Value=0.05
  k Cp : Gain
  lambda calc : Product  Inputs=*/
  max W : MinMax  Function=max  Inputs=2
  max v : MinMax  Function=max  Inputs=2
  v min : Constant  Value=0.1
  Tw : Outport
  Cp : Outport  Port=2
  lambda : Outport  Port=3
  wires:
  v min/1 -> max v/2
  W/1 -> max W/1
  W min/1 -> max W/2
  v/1 -> max v/1
  lambda calc/1 -> Cp(lambda)/1, lambda/1
  max W/1 -> Cp v3 over W/5, R/1
  R/1 -> lambda calc/1
  max v/1 -> Cp v3 over W/2, Cp v3 over W/3, Cp v3 over W/4, lambda calc/2
  Cp(lambda)/1 -> k Cp/1
  k Cp/1 -> Cp/1, Cp v3 over W/1
  Cp v3 over W/1 -> 0.5 rho pi R^2/1
  0.5 rho pi R^2/1 -> Tw/1
